simulink model "PMLSM_PI_FOC_Float_Baseline"  (R2026b)
settings: Solver=FixedStepDiscrete  StopTime=M1A_StopTime_s  FixedStep=Ts_Plant
InitFcn:
  | m1a_require_float_init(bdroot);
values from neighbouring files (symbols this model uses):
  Alignment_Enable = 0    [init_PMLSM_PI_FOC_Float_Baseline.m]
  Hold_Ticks = 30000    [init_PMLSM_PI_FOC_Float_Baseline.m]
  Host_AutoStart_EN = 1    [init_PMLSM_PI_FOC_Float_Baseline.m]
  Host_Close_Loop_EN = 1    [init_PMLSM_PI_FOC_Float_Baseline.m]
  Host_Id_A = 0    [init_PMLSM_PI_FOC_Float_Baseline.m]
  Host_Iq_A = 0    [init_PMLSM_PI_FOC_Float_Baseline.m]
  Host_Iq_Test_Mode = 0    [init_PMLSM_PI_FOC_Float_Baseline.m]
  Host_Load_N = 0    [init_PMLSM_PI_FOC_Float_Baseline.m]
  Host_Move_Request = 0    [init_PMLSM_PI_FOC_Float_Baseline.m]
  Host_PI_Reset_EN = 0    [init_PMLSM_PI_FOC_Float_Baseline.m]
  Host_Position_Loop_EN = 1    [init_PMLSM_PI_FOC_Float_Baseline.m]
  Host_PWM_EN = 1    [init_PMLSM_PI_FOC_Float_Baseline.m]
  Host_Ready_Ticks = 5    [init_PMLSM_PI_FOC_Float_Baseline.m]
  Host_Replay_EN = 0    [init_PMLSM_PI_FOC_Float_Baseline.m]
  Host_Speed_mmps = 0    [init_PMLSM_PI_FOC_Float_Baseline.m]
  Host_Speed_Ramp_s = 0.1    [init_PMLSM_PI_FOC_Float_Baseline.m]
  Host_Start_s = 0.05    [init_PMLSM_PI_FOC_Float_Baseline.m]
  Host_Target_mm = 10    [init_PMLSM_PI_FOC_Float_Baseline.m]
  Host_Traj_Amax = 100    [init_PMLSM_PI_FOC_Float_Baseline.m]
  Host_Traj_Jmax = 1000    [init_PMLSM_PI_FOC_Float_Baseline.m]
  Host_Traj_Vmax = 10    [init_PMLSM_PI_FOC_Float_Baseline.m]
  Id_Init_Step = Id_Init_Target/Ramp_Ticks    (= 5e-05)    [init_PMLSM_PI_FOC_Float_Baseline.m]
  Id_Init_Target = 0.5    [init_PMLSM_PI_FOC_Float_Baseline.m]
  Id_Release_Ramp_Ticks = 2000    [init_PMLSM_PI_FOC_Float_Baseline.m]
  Init_Reset = 0    [init_PMLSM_PI_FOC_Float_Baseline.m]
  Init_Start = 0    [init_PMLSM_PI_FOC_Float_Baseline.m]
  Iq_int_limit = 0.5    [init_PMLSM_PI_FOC_Float_Baseline.m]
  Kaw_d = Tuning_Gains.Kaw_d    [init_PMLSM_PI_FOC_Float_Baseline.m]
  Kaw_q = Tuning_Gains.Kaw_q    [init_PMLSM_PI_FOC_Float_Baseline.m]
  Kaw_s = Tuning_Gains.Kaw_s    [init_PMLSM_PI_FOC_Float_Baseline.m]
  Ki_ACR = Tuning_Gains.Ki_ACR    [init_PMLSM_PI_FOC_Float_Baseline.m]
  Ki_ASR = Tuning_Gains.Ki_ASR    [init_PMLSM_PI_FOC_Float_Baseline.m]
  Kp_ACR = Tuning_Gains.Kp_ACR    [init_PMLSM_PI_FOC_Float_Baseline.m]
  Kp_ASR = Tuning_Gains.Kp_ASR    [init_PMLSM_PI_FOC_Float_Baseline.m]
  Kp_pos = Tuning_Gains.Kp_pos    [init_PMLSM_PI_FOC_Float_Baseline.m]
  M1A_PWM_Update_Delay_s = T_pwm/2    (= 5e-05)    [init_PMLSM_PI_FOC_Float_Baseline.m]
  PMLSM_Bv_N_per_mps = 0    [init_PMLSM_PI_FOC_Float_Baseline.m]
  PMLSM_deadtime_current_eps_A = 1e-4    (= 0.0001)    [init_PMLSM_PI_FOC_Float_Baseline.m]
  PMLSM_deadtime_ratio = PMLSM_deadtime_s/T_pwm    (= 0.01)    [init_PMLSM_PI_FOC_Float_Baseline.m]
  PMLSM_Fc_N = 0    [init_PMLSM_PI_FOC_Float_Baseline.m]
  PMLSM_Kf_peak_N_per_Apeak = 31.4/sqrt(2)    [init_PMLSM_PI_FOC_Float_Baseline.m]
  PMLSM_Ld_H = 1.745e-3    (= 0.001745)    [init_PMLSM_PI_FOC_Float_Baseline.m]
  PMLSM_Lq_H = PMLSM_Ld_H    (= 0.001745)    [init_PMLSM_PI_FOC_Float_Baseline.m]
  PMLSM_M_kg = 0.91    [init_PMLSM_PI_FOC_Float_Baseline.m]
  PMLSM_psi_f_Wb = 0.141    [init_PMLSM_PI_FOC_Float_Baseline.m]
  PMLSM_Rs_ohm = 2.37    [init_PMLSM_PI_FOC_Float_Baseline.m]
  PMLSM_tau_NN_m = 0.06    [init_PMLSM_PI_FOC_Float_Baseline.m]
  PMLSM_theta_offset_rad = 0    [init_PMLSM_PI_FOC_Float_Baseline.m]
  PMLSM_Ts_s = Ts_Plant    (= 1e-06)    [init_PMLSM_PI_FOC_Float_Baseline.m]
  PMLSM_v_eps_mps = 1e-3    (= 0.001)    [init_PMLSM_PI_FOC_Float_Baseline.m]
  Pos_deadband = 0.02    [init_PMLSM_PI_FOC_Float_Baseline.m]
  Ramp_Ticks = 10000    [init_PMLSM_PI_FOC_Float_Baseline.m]
  Simulation_Travel_Fault = 0    [init_PMLSM_PI_FOC_Float_Baseline.m]
  Speed_loop_Iq_Limit = 1    [init_PMLSM_PI_FOC_Float_Baseline.m]
  T_pwm = 1e-4    (= 0.0001)    [init_PMLSM_PI_FOC_Float_Baseline.m]
  Tau_e_mm = PMLSM_tau_NN_m*1000    (= 60)    [init_PMLSM_PI_FOC_Float_Baseline.m]
  theta_align_const = 0    [init_PMLSM_PI_FOC_Float_Baseline.m]
  Theta_Offset_Fine = 0    [init_PMLSM_PI_FOC_Float_Baseline.m]
  Ts = Ts_ACR    (= 0.0001)    [init_PMLSM_PI_FOC_Float_Baseline.m]
  Ts_ACR = T_pwm    (= 0.0001)    [init_PMLSM_PI_FOC_Float_Baseline.m]
  Ts_ASR = 10*Ts_ACR    (= 0.001)    [init_PMLSM_PI_FOC_Float_Baseline.m]
  Ts_Plant = 1e-6    (= 1e-06)    [init_PMLSM_PI_FOC_Float_Baseline.m]
  Ts_POS = 10*Ts_ASR    (= 0.01)    [init_PMLSM_PI_FOC_Float_Baseline.m]
  Udc = 48    [init_PMLSM_PI_FOC_Float_Baseline.m]
  v_ff_eps = 0.5    [init_PMLSM_PI_FOC_Float_Baseline.m]
  v_over_eps = 3    [init_PMLSM_PI_FOC_Float_Baseline.m]
  V_pos_max_mmps = 20    [init_PMLSM_PI_FOC_Float_Baseline.m]
  v_ref_max = 20    [init_PMLSM_PI_FOC_Float_Baseline.m]
  v_ref_set_step_dn = v_ref_set_rate_dn*Ts_ACR    (= 0.005)    [init_PMLSM_PI_FOC_Float_Baseline.m]
  v_ref_set_step_up = v_ref_set_rate_up*Ts_ACR    (= 0.005)    [init_PMLSM_PI_FOC_Float_Baseline.m]
  v_ref_zero_eps = 0    [init_PMLSM_PI_FOC_Float_Baseline.m]
undefined symbols (not defined in the file or in its folder): DiscIntNeverNeededParam, Iq_fric_run, Iq_fric_start, v_stick_off, v_stick_on
libraries: simulink x7, mcbeeMathTransformLib x2
(part 1 of 2)
settings Model: Creator=lww  LastModifiedBy=lww
settings DataIOCC: SaveOutput=off  SaveTime=off

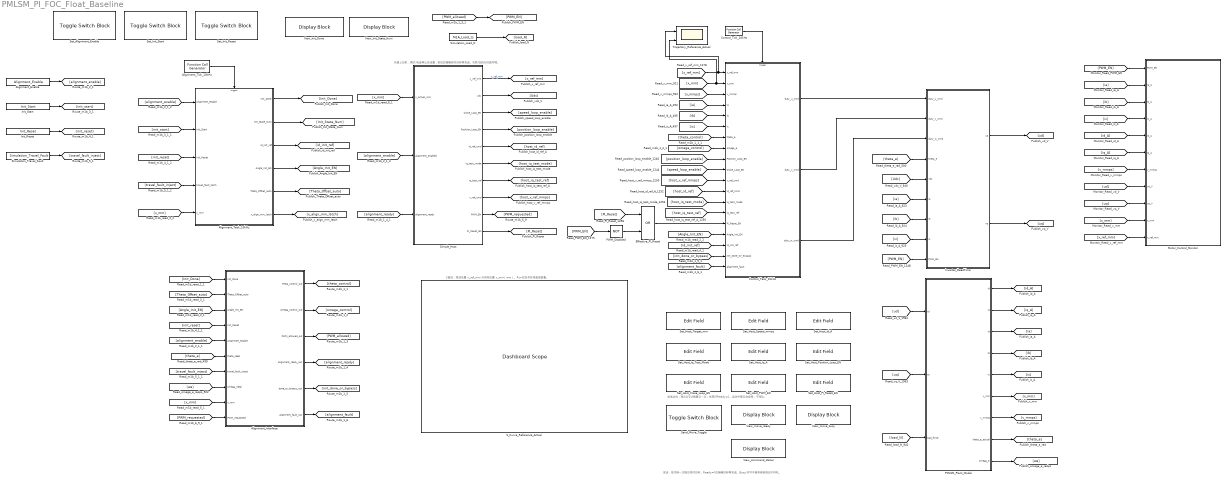
== system PMLSM_PI_FOC_Float_Baseline ==
  note: 仿真上位机：模式/轨迹停止后设置；到位后编辑绝对目标再发送。负载/母线为仿真环境。
  note: S曲线：规划位置 x_ref_mm 与实际位置 x_mm（mm）。Run后在本区域直接查看。
  note: 发送点位：每次0/1切换提交一次；先等待Ready=1，运动中提交会拒绝，不排队。
  note: 发送：每切换一次提交绝对目标；Ready=1后编辑目标再发送。Busy/对齐中请求被拒绝且不排队。
  Alignment_Enable : Constant  Value=Alignment_Enable  OutDataTypeStr=double  SampleTime=Ts_ACR
  Alignment_Interface : Subsystem
  Alignment_Task_10kHz : Subsystem
  Alignment_Tick_10kHz : FunctionCallGenerator  Priority=-100  SampleTime=Ts
  Control_Task_10kHz : Subsystem
  Control_Tick_10kHz : FunctionCallGenerator  Priority=100  SampleTime=Ts
  Effective_PI_Reset : Logic  Operator=OR  AllPortsSameDT=off  OutDataTypeStr=boolean
  Init_Reset : Constant  Value=Init_Reset  SampleTime=Ts_ACR
  Init_Start : Constant  Value=Init_Start  SampleTime=Ts_ACR
  Inverter_DeadTime : Subsystem
  Motor_Control_Monitor : Subsystem
  PMLSM_Plant_Model : Subsystem
  PWM_Disabled : Logic  Operator=NOT  AllPortsSameDT=off  OutDataTypeStr=boolean
  S_Curve_Reference_Actual : DashboardScope  FontColor=[0.0, 0.0, 0.0]
  Send_Move_Toggle : ToggleSwitchBlock
  Set_Alignment_Enable : ToggleSwitchBlock
  Set_Host_Close_Loop_EN : EditField  ShowInitialText=on  Alignment=Center
  Set_Host_Id_A : EditField  ShowInitialText=on  Alignment=Center
  Set_Host_Iq_A : EditField  ShowInitialText=on  Alignment=Center
  Set_Host_Iq_Test_Mode : EditField  ShowInitialText=on  Alignment=Center
  Set_Host_PI_Reset_EN : EditField  ShowInitialText=on  Alignment=Center
  Set_Host_PWM_EN : EditField  ShowInitialText=on  Alignment=Center
  Set_Host_Position_Loop_EN : EditField  ShowInitialText=on  Alignment=Center
  Set_Host_Speed_mmps : EditField  ShowInitialText=on  Alignment=Center
  Set_Host_Target_mm : EditField  ShowInitialText=on  Alignment=Center
  Set_Init_Reset : ToggleSwitchBlock
  Set_Init_Start : ToggleSwitchBlock
  Simple_Host : Subsystem
  Simulation_Load_N : FromWorkspace  VariableName=M1A_Load_ts  SampleTime=Ts_Plant  Interpolate=off  OutputAfterFinalValue=Holding final value
  Simulation_Travel_Fault : Constant  Value=Simulation_Travel_Fault  OutDataTypeStr=double  SampleTime=Ts_ACR
  Trajectory_Reference_Actual : Scope  NumInputPorts=2
      settings: ActiveDisplayYMinimum=0.99182264665726316  ActiveDisplayYMaximum=1.0007838303678565
  View_Init_Done : DisplayBlock  Transparency=1  GridColor=[0.502, 0.502, 0.502]
  View_Init_State_Num : DisplayBlock  Transparency=1  GridColor=[0.502, 0.502, 0.502]
  View_command_status : DisplayBlock  Transparency=1  GridColor=[0.502, 0.502, 0.502]
  View_move_busy : DisplayBlock  Transparency=1  GridColor=[0.502, 0.502, 0.502]
  View_move_ready : DisplayBlock  Transparency=1  GridColor=[0.502, 0.502, 0.502]
  wires:
  [PWM_EN] -> PWM_Disabled/1
  PWM_Disabled/1 -> Effective_PI_Reset/2
  Effective_PI_Reset/1 -> Control_Task_10kHz/15(PI_Reset_EN)
  [speed_loop_enable] -> Control_Task_10kHz/10(Close_Loop_EN)
  [position_loop_enable] -> Control_Task_10kHz/9(Position_Loop_EN)
  [host_v_ref_mmps] -> Control_Task_10kHz/11(v_ref_cmd)
  [host_id_ref] -> Control_Task_10kHz/12(id_ref_cmd)
  [host_iq_test_mode] -> Control_Task_10kHz/13(iq_test_mode)
  [host_iq_test_ref] -> Control_Task_10kHz/14(iq_test_ref)
  [PI_Reset] -> Effective_PI_Reset/1
  [x_mm] -> Trajectory_Reference_Actual/2, Control_Task_10kHz/2(x_mm)
  [v_mmps] -> Control_Task_10kHz/3(v_mmps)
  [ia] -> Control_Task_10kHz/4(ia)
  [ib] -> Control_Task_10kHz/5(ib)
  [ic] -> Control_Task_10kHz/6(ic)
  [x_ref_mm] -> Trajectory_Reference_Actual/1, Control_Task_10kHz/1(x_ref_mm)
  PMLSM_Plant_Model/6(x_mm) -> [x_mm]
  PMLSM_Plant_Model/7(v_mmps) -> [v_mmps]
  PMLSM_Plant_Model/3(ia) -> [ia]
  PMLSM_Plant_Model/4(ib) -> [ib]
  PMLSM_Plant_Model/5(ic) -> [ic]
  PMLSM_Plant_Model/8(theta_e_actual) -> [theta_e]
  PMLSM_Plant_Model/9(omega_e) -> [we]
  PMLSM_Plant_Model/1(id) -> [id_A]
  PMLSM_Plant_Model/2(iq) -> [iq_A]
  [load_N] -> PMLSM_Plant_Model/3(load_force)
  [uq] -> PMLSM_Plant_Model/2(vq)
  [ud] -> PMLSM_Plant_Model/1(vd)
  [ic] -> Inverter_DeadTime/8(ic)
  [ib] -> Inverter_DeadTime/7(ib)
  [ia] -> Inverter_DeadTime/6(ia)
  [theta_e] -> Inverter_DeadTime/4(theta_e)
  [Udc] -> Inverter_DeadTime/5(vdc)
  Inverter_DeadTime/1(vd) -> [ud]
  Inverter_DeadTime/2(vq) -> [uq]
  [PWM_EN] -> Inverter_DeadTime/9(PWM_EN)
  Control_Task_10kHz/1(duty_u_cmd) -> Inverter_DeadTime/1(duty_u_cmd)
  Control_Task_10kHz/2(duty_v_cmd) -> Inverter_DeadTime/2(duty_v_cmd)
  Control_Task_10kHz/3(duty_w_cmd) -> Inverter_DeadTime/3(duty_w_cmd)
  Simulation_Load_N/1 -> [load_N]
  Simple_Host/1(x_ref_mm) -> [x_ref_mm]  "x_ref_mm"
  Simple_Host/2(vdc) -> [Udc]
  Simple_Host/3(Close_Loop_EN) -> [speed_loop_enable]
  Simple_Host/4(Position_Loop_EN) -> [position_loop_enable]
  Simple_Host/5(id_ref_cmd) -> [host_id_ref]
  Simple_Host/6(iq_test_mode) -> [host_iq_test_mode]
  Simple_Host/7(iq_test_ref) -> [host_iq_test_ref]
  Simple_Host/8(v_ref_cmd) -> [host_v_ref_mmps]
  Simple_Host/10(PI_Reset_EN) -> [PI_Reset]
  [PWM_EN] -> Motor_Control_Monitor/1(PWM_EN)
  [ia] -> Motor_Control_Monitor/2(ia_A)
  [ib] -> Motor_Control_Monitor/3(ib_A)
  [ic] -> Motor_Control_Monitor/4(ic_A)
  [id_A] -> Motor_Control_Monitor/5(id_A)
  [iq_A] -> Motor_Control_Monitor/6(iq_A)
  [v_mmps] -> Motor_Control_Monitor/7(v_mmps)
  [ud] -> Motor_Control_Monitor/8(vd_V)
  [uq] -> Motor_Control_Monitor/9(vq_V)
  [x_mm] -> Motor_Control_Monitor/10(x_mm)
  [x_ref_mm] -> Motor_Control_Monitor/11(x_ref_mm)
  Alignment_Task_10kHz/1(Init_Done) -> [Init_Done]
  Alignment_Task_10kHz/2(Init_State_Num) -> [Init_State_Num]
  Alignment_Task_10kHz/3(id_init_ref) -> [id_init_ref]
  Alignment_Task_10kHz/4(Angle_Init_EN) -> [Angle_Init_EN]
  Alignment_Task_10kHz/5(Theta_Offset_auto) -> [Theta_Offset_auto]
  Alignment_Task_10kHz/6(x_align_mm_latch) -> [x_align_mm_latch]
  Alignment_Tick_10kHz/1 -> Alignment_Task_10kHz/Trigger
  Control_Tick_10kHz/1 -> Control_Task_10kHz/Trigger
  [theta_e] -> Alignment_Interface/6(theta_ideal)
  [we] -> Alignment_Interface/8(omega_ideal)
  Alignment_Interface/1(theta_control_out) -> [theta_control]
  [theta_control] -> Control_Task_10kHz/7(theta_e)
  Alignment_Interface/2(omega_control_out) -> [omega_control]
  [omega_control] -> Control_Task_10kHz/8(omega_e)
  Alignment_Interface/3(PWM_allowed_out) -> [PWM_allowed]
  [PWM_allowed] -> [PWM_EN]
  Alignment_Interface/4(alignment_ready_out) -> [alignment_ready]
  [alignment_ready] -> Simple_Host/3(alignment_ready)
  Alignment_Interface/5(done_or_bypass_out) -> [init_done_or_bypass]
  [init_done_or_bypass] -> Control_Task_10kHz/18(Init_Done_Or_Bypass)
  Alignment_Interface/6(alignment_fault_out) -> [alignment_fault]
  [alignment_fault] -> Control_Task_10kHz/19(alignment_fault)
  Alignment_Enable/1 -> [alignment_enable]
  [alignment_enable] -> Alignment_Interface/5(Alignment_Enable)
  [alignment_enable] -> Alignment_Task_10kHz/1(Alignment_Enable)
  [alignment_enable] -> Simple_Host/2(alignment_enabled)
  Init_Start/1 -> [init_start]
  [init_start] -> Alignment_Task_10kHz/2(Init_Start)
  Init_Reset/1 -> [init_reset]
  [init_reset] -> Alignment_Interface/4(Init_Reset)
  [init_reset] -> Alignment_Task_10kHz/3(Init_Reset)
  Simulation_Travel_Fault/1 -> [travel_fault_inject]
  [travel_fault_inject] -> Alignment_Interface/7(travel_fault_inject)
  [travel_fault_inject] -> Alignment_Task_10kHz/4(travel_fault_latch)
  Simple_Host/9(PWM_EN) -> [PWM_requested]
  [PWM_requested] -> Alignment_Interface/10(PWM_requested)
  [Init_Done] -> Alignment_Interface/1(Init_Done)
  [Angle_Init_EN] -> Alignment_Interface/3(Angle_Init_EN)
  [Angle_Init_EN] -> Control_Task_10kHz/16(Angle_Init_EN)
  [Theta_Offset_auto] -> Alignment_Interface/2(Theta_Offset_auto)
  [id_init_ref] -> Control_Task_10kHz/17(id_init_ref)
  [x_mm] -> Alignment_Interface/9(x_mm)
  [x_mm] -> Alignment_Task_10kHz/5(x_mm)
  [x_mm] -> Simple_Host/1(x_actual_mm)

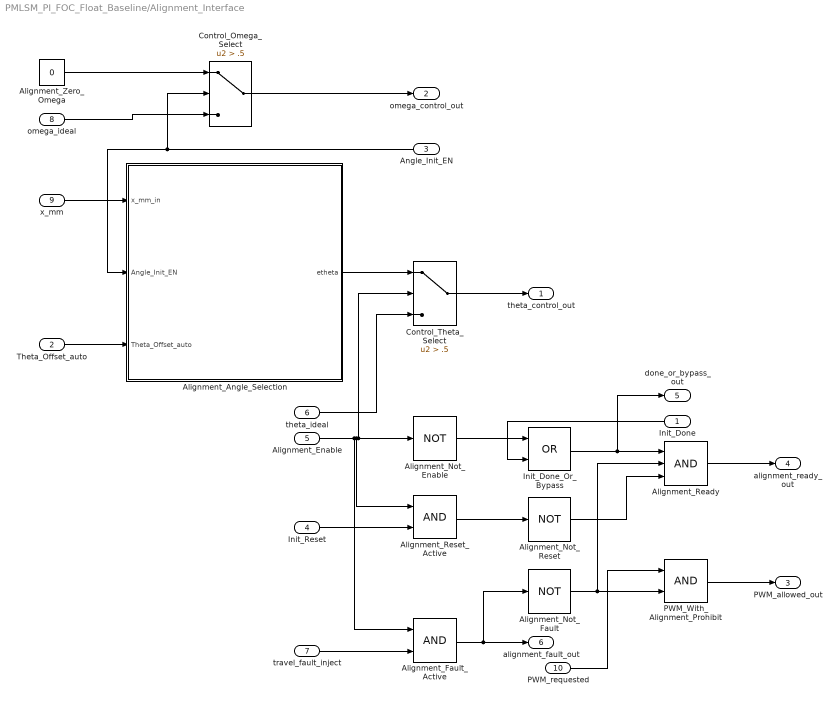
== system PMLSM_PI_FOC_Float_Baseline/Alignment_Interface ==
  Init_Done : Inport
  Theta_Offset_auto : Inport  Port=2
  Angle_Init_EN : Inport  Port=3
  Init_Reset : Inport  Port=4
  Alignment_Enable : Inport  Port=5
  theta_ideal : Inport  Port=6
  travel_fault_inject : Inport  Port=7
  omega_ideal : Inport  Port=8
  x_mm : Inport  Port=9
  PWM_requested : Inport  Port=10
  Alignment_Angle_Selection : Subsystem
  Alignment_Fault_Active : Logic  AllPortsSameDT=off  OutDataTypeStr=boolean
  Alignment_Not_Enable : Logic  Operator=NOT  AllPortsSameDT=off  OutDataTypeStr=boolean
  Alignment_Not_Fault : Logic  Operator=NOT  AllPortsSameDT=off  OutDataTypeStr=boolean
  Alignment_Not_Reset : Logic  Operator=NOT  AllPortsSameDT=off  OutDataTypeStr=boolean
  Alignment_Ready : Logic  Inputs=3  AllPortsSameDT=off  OutDataTypeStr=boolean
  Alignment_Reset_Active : Logic  AllPortsSameDT=off  OutDataTypeStr=boolean
  Alignment_Zero_Omega : Constant  Value=0
  Control_Omega_Select : Switch  Criteria=u2 > Threshold  Threshold=.5
  Control_Theta_Select : Switch  Criteria=u2 > Threshold  Threshold=.5
  Init_Done_Or_Bypass : Logic  Operator=OR  AllPortsSameDT=off  OutDataTypeStr=boolean
  PWM_With_Alignment_Prohibit : Logic  AllPortsSameDT=off  OutDataTypeStr=boolean
  theta_control_out : Outport
  omega_control_out : Outport  Port=2
  PWM_allowed_out : Outport  Port=3
  alignment_ready_out : Outport  Port=4
  done_or_bypass_out : Outport  Port=5
  alignment_fault_out : Outport  Port=6
  wires:
  Init_Done/1 -> Init_Done_Or_Bypass/2
  Alignment_Zero_Omega/1 -> Control_Omega_Select/1
  omega_ideal/1 -> Control_Omega_Select/3
  Alignment_Not_Enable/1 -> Init_Done_Or_Bypass/1
  Alignment_Enable/1 -> Alignment_Not_Enable/1, Control_Theta_Select/2, Alignment_Reset_Active/1, Alignment_Fault_Active/1
  x_mm/1 -> Alignment_Angle_Selection/1(x_mm_in)
  Alignment_Ready/1 -> alignment_ready_out/1
  Alignment_Angle_Selection/1(etheta) -> Control_Theta_Select/1
  Theta_Offset_auto/1 -> Alignment_Angle_Selection/3(Theta_Offset_auto)
  Control_Omega_Select/1 -> omega_control_out/1
  theta_ideal/1 -> Control_Theta_Select/3
  Init_Reset/1 -> Alignment_Reset_Active/2
  travel_fault_inject/1 -> Alignment_Fault_Active/2
  Angle_Init_EN/1 -> Control_Omega_Select/2, Alignment_Angle_Selection/2(Angle_Init_EN)
  Control_Theta_Select/1 -> theta_control_out/1
  Alignment_Reset_Active/1 -> Alignment_Not_Reset/1
  Alignment_Fault_Active/1 -> Alignment_Not_Fault/1, alignment_fault_out/1
  Init_Done_Or_Bypass/1 -> done_or_bypass_out/1, Alignment_Ready/1
  Alignment_Not_Reset/1 -> Alignment_Ready/3
  Alignment_Not_Fault/1 -> Alignment_Ready/2, PWM_With_Alignment_Prohibit/2
  PWM_requested/1 -> PWM_With_Alignment_Prohibit/1
  PWM_With_Alignment_Prohibit/1 -> PWM_allowed_out/1

== system PMLSM_PI_FOC_Float_Baseline/Alignment_Task_10kHz ==
  Alignment_Enable : Inport
  Init_Start : Inport  Port=2
  Init_Reset : Inport  Port=3
  travel_fault_latch : Inport  Port=4
  x_mm : Inport  Port=5
  Tick : TriggerPort  TriggerType=function-call  VariantControl=(inherit)
  Enabled_Original_MIL : Subsystem
  Init_Done : Outport
  Init_State_Num : Outport  Port=2
  id_init_ref : Outport  Port=3
  Angle_Init_EN : Outport  Port=4
  Theta_Offset_auto : Outport  Port=5
  x_align_mm_latch : Outport  Port=6
  wires:
  Alignment_Enable/1 -> Enabled_Original_MIL/Enable
  Enabled_Original_MIL/2(Init_State_Num) -> Init_State_Num/1
  Init_Start/1 -> Enabled_Original_MIL/1(Init_Start)
  Enabled_Original_MIL/3(id_init_ref) -> id_init_ref/1
  Init_Reset/1 -> Enabled_Original_MIL/2(Init_Reset)
  travel_fault_latch/1 -> Enabled_Original_MIL/3(travel_fault_latch)
  x_mm/1 -> Enabled_Original_MIL/4(x_mm)
  Enabled_Original_MIL/1(Init_Done) -> Init_Done/1
  Enabled_Original_MIL/4(Angle_Init_EN) -> Angle_Init_EN/1
  Enabled_Original_MIL/5(Theta_Offset_auto) -> Theta_Offset_auto/1
  Enabled_Original_MIL/6(x_align_mm_latch) -> x_align_mm_latch/1

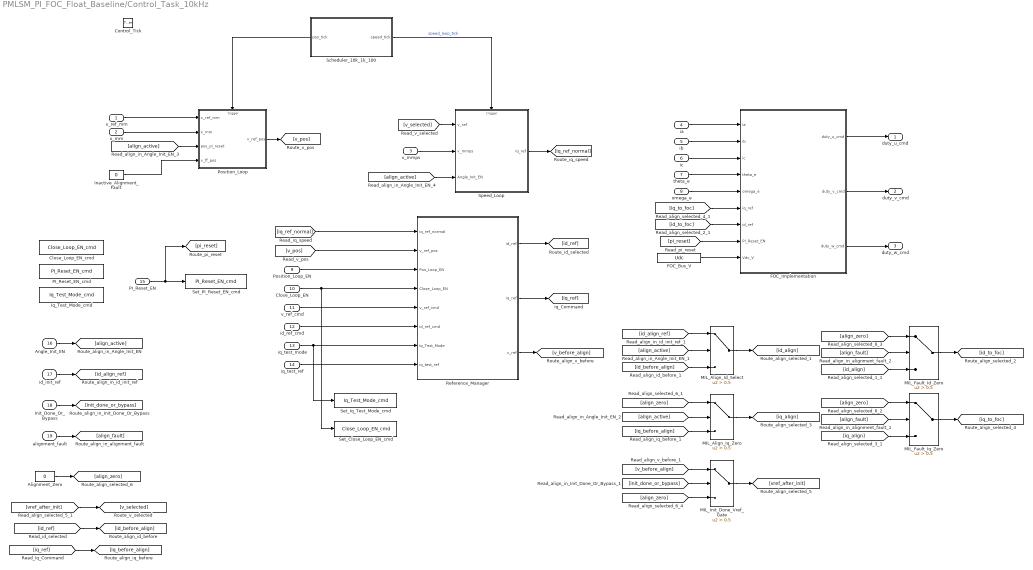
== system PMLSM_PI_FOC_Float_Baseline/Control_Task_10kHz ==
  x_ref_mm : Inport
  x_mm : Inport  Port=2
  v_mmps : Inport  Port=3
  ia : Inport  Port=4
  ib : Inport  Port=5
  ic : Inport  Port=6
  theta_e : Inport  Port=7
  omega_e : Inport  Port=8
  Position_Loop_EN : Inport  Port=9
  Close_Loop_EN : Inport  Port=10
  v_ref_cmd : Inport  Port=11
  id_ref_cmd : Inport  Port=12
  iq_test_mode : Inport  Port=13
  iq_test_ref : Inport  Port=14
  PI_Reset_EN : Inport  Port=15
  Angle_Init_EN : Inport  Port=16
  id_init_ref : Inport  Port=17
  Init_Done_Or_Bypass : Inport  Port=18
  alignment_fault : Inport  Port=19
  Control_Tick : TriggerPort  TriggerType=function-call  VariantControl=(inherit)  PortDimensions=1
  Alignment_Zero : Constant  Value=0
  Close_Loop_EN_cmd : DataStoreMemory  DataStoreName=Close_Loop_EN_cmd  WriteAfterWriteMsg=warning  InitialValue=1  ShowAdditionalParam=off
  FOC_Bus_V : Constant  Value=Udc  SampleTime=-1
  FOC_Implementation : Subsystem  Variant=on  EmptyChoice=on
  Inactive_Alignment_Fault : Constant  Value=0
  Iq_Test_Mode_cmd : DataStoreMemory  DataStoreName=Iq_Test_Mode_cmd  WriteAfterWriteMsg=warning  ShowAdditionalParam=off
  MIL_Align_Id_Select : Switch  Criteria=u2 > Threshold  Threshold=0.5  SaturateOnIntegerOverflow=off  InputSameDT=off
  MIL_Align_Iq_Zero : Switch  Criteria=u2 > Threshold  Threshold=0.5  SaturateOnIntegerOverflow=off  InputSameDT=off
  MIL_Fault_Id_Zero : Switch  Criteria=u2 > Threshold  Threshold=0.5  SaturateOnIntegerOverflow=off  InputSameDT=off
  MIL_Fault_Iq_Zero : Switch  Criteria=u2 > Threshold  Threshold=0.5  SaturateOnIntegerOverflow=off  InputSameDT=off
  MIL_Init_Done_Vref_Gate : Switch  Criteria=u2 > Threshold  Threshold=0.5  SaturateOnIntegerOverflow=off  InputSameDT=off
  PI_Reset_EN_cmd : DataStoreMemory  DataStoreName=PI_Reset_EN_cmd  WriteAfterWriteMsg=warning  ShowAdditionalParam=off
  Position_Loop : Subsystem  TreatAsAtomicUnit=on
  Reference_Manager : Subsystem
  Scheduler_10k_1k_100 : Subsystem
      settings: PortSchema="{\"entries\":[{\"content\":{\"sides\":[{\"content\":{\"connectorIds\":[\"Out2\"]},\"type\":\"ConnectorPlacement.EquallySpacedRectSide\",\"uuid\":\"7a2cd2ad-1b6d-4ced-b4c0-dea2e76e4441\"},{\"content\":{\"connectorIds\":[\"Out1\"],\"side\":\"RIGHT\"},\"type\":\"ConnectorPlacement.EquallySpacedRectSide\",\"uuid\":\"f7db3b94-1126-4089-83bd-8e57d20e6fd7\"},{\"content\":{\"side\":\"TOP\"},\"type\":\"ConnectorPlacement.EquallySpacedRectSide\",\"uuid\":\"9153f6b5-22af-48be-92c0-68be43f93648\"}]},\"type\":\"ConnectorPlacement.EquallySpacedConnector\",\"uuid\":\"029fb485-bddc-4cd2-9c64-7547c8dffd2b\"}],\"packageUris\":[\"http://schema.mathworks.com/mf0/Connector/R2020b\"],\"version\":\"1.0\"}"
  Set_Close_Loop_EN_cmd : DataStoreWrite  Priority=-10  DataStoreName=Close_Loop_EN_cmd  IndexOptions=Index vector (dialog)  Indices=1  OutputSizes=1
  Set_Iq_Test_Mode_cmd : DataStoreWrite  Priority=-10  DataStoreName=Iq_Test_Mode_cmd  IndexOptions=Index vector (dialog)  Indices=1  OutputSizes=1
  Set_PI_Reset_EN_cmd : DataStoreWrite  Priority=-10  DataStoreName=PI_Reset_EN_cmd  IndexOptions=Index vector (dialog)  Indices=1  OutputSizes=1
  Speed_Loop : Subsystem  TreatAsAtomicUnit=on
  duty_u_cmd : Outport
  duty_v_cmd : Outport  Port=2
  duty_w_cmd : Outport  Port=3
  wires:
  iq_test_ref/1 -> Reference_Manager/8(iq_test_ref)
  id_ref_cmd/1 -> Reference_Manager/6(id_ref_cmd)
  v_ref_cmd/1 -> Reference_Manager/5(v_ref_cmd)
  Position_Loop_EN/1 -> Reference_Manager/3(Pos_Loop_EN)
  [v_selected] -> Speed_Loop/1(v_ref)
  [iq_ref_normal] -> Reference_Manager/1(iq_ref_normal)
  [v_pos] -> Reference_Manager/2(v_ref_pos)
  Inactive_Alignment_Fault/1 -> Position_Loop/4(v_ff_pos)
  Speed_Loop/1(iq_ref) -> [iq_ref_normal]
  Position_Loop/1(v_ref_pos) -> [v_pos]
  x_mm/1 -> Position_Loop/2(x_mm)
  x_ref_mm/1 -> Position_Loop/1(x_ref_mm)
  Scheduler_10k_1k_100/1(speed_tick) -> Speed_Loop/Trigger  "speed_loop_tick"
  Scheduler_10k_1k_100/2(pos_tick) -> Position_Loop/Trigger
  PI_Reset_EN/1 -> [pi_reset], Set_PI_Reset_EN_cmd/1
  iq_test_mode/1 -> Set_Iq_Test_Mode_cmd/1, Reference_Manager/7(Iq_Test_Mode)
  Close_Loop_EN/1 -> Set_Close_Loop_EN_cmd/1, Reference_Manager/4(Close_Loop_EN)
  v_mmps/1 -> Speed_Loop/2(v_mmps)
  Reference_Manager/1(id_ref) -> [id_ref]
  Reference_Manager/2(iq_ref) -> [iq_ref]
  MIL_Align_Id_Select/1 -> [id_align]
  [id_align] -> MIL_Fault_Id_Zero/3
  MIL_Fault_Id_Zero/1 -> [id_to_foc]
  MIL_Align_Iq_Zero/1 -> [iq_align]
  [iq_align] -> MIL_Fault_Iq_Zero/3
  MIL_Fault_Iq_Zero/1 -> [iq_to_foc]
  MIL_Init_Done_Vref_Gate/1 -> [vref_after_init]
  [vref_after_init] -> [v_selected]
  Alignment_Zero/1 -> [align_zero]
  [align_zero] -> MIL_Align_Iq_Zero/1
  [align_zero] -> MIL_Fault_Iq_Zero/1
  [align_zero] -> MIL_Fault_Id_Zero/1
  [align_zero] -> MIL_Init_Done_Vref_Gate/3
  Angle_Init_EN/1 -> [align_active]
  [align_active] -> MIL_Align_Id_Select/2
  [align_active] -> MIL_Align_Iq_Zero/2
  [align_active] -> Position_Loop/3(pos_pi_reset)
  [align_active] -> Speed_Loop/3(Angle_Init_EN)
  id_init_ref/1 -> [id_align_ref]
  [id_align_ref] -> MIL_Align_Id_Select/1
  Init_Done_Or_Bypass/1 -> [init_done_or_bypass]
  [init_done_or_bypass] -> MIL_Init_Done_Vref_Gate/2
  alignment_fault/1 -> [align_fault]
  [align_fault] -> MIL_Fault_Iq_Zero/2
  [align_fault] -> MIL_Fault_Id_Zero/2
  [id_ref] -> [id_before_align]
  [id_before_align] -> MIL_Align_Id_Select/3
  [iq_ref] -> [iq_before_align]
  [iq_before_align] -> MIL_Align_Iq_Zero/3
  Reference_Manager/3(v_ref) -> [v_before_align]
  [v_before_align] -> MIL_Init_Done_Vref_Gate/1
  ia/1 -> FOC_Implementation/1(ia)
  ib/1 -> FOC_Implementation/2(ib)
  ic/1 -> FOC_Implementation/3(ic)
  theta_e/1 -> FOC_Implementation/4(theta_e)
  omega_e/1 -> FOC_Implementation/5(omega_e)
  [iq_to_foc] -> FOC_Implementation/6(iq_ref)
  [id_to_foc] -> FOC_Implementation/7(id_ref)
  [pi_reset] -> FOC_Implementation/8(PI_Reset_EN)
  FOC_Implementation/1(duty_u_cmd) -> duty_u_cmd/1
  FOC_Implementation/2(duty_v_cmd) -> duty_v_cmd/1
  FOC_Implementation/3(duty_w_cmd) -> duty_w_cmd/1
  FOC_Bus_V/1 -> FOC_Implementation/9(Vdc_V)

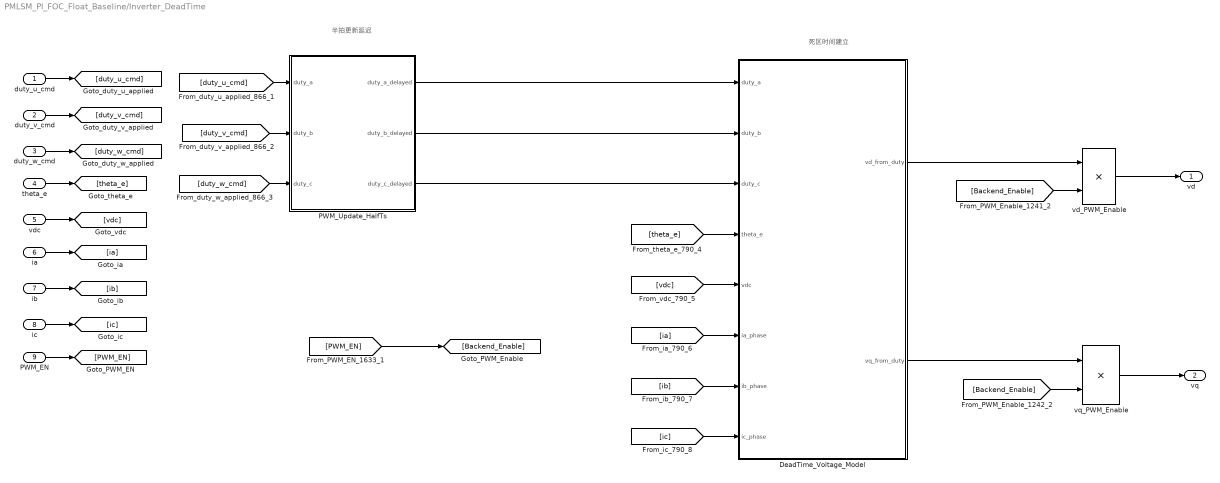
== system PMLSM_PI_FOC_Float_Baseline/Inverter_DeadTime ==
  note: 死区时间建立
  note: 半拍更新延迟
  duty_u_cmd : Inport
  duty_v_cmd : Inport  Port=2
  duty_w_cmd : Inport  Port=3
  theta_e : Inport  Port=4
  vdc : Inport  Port=5
  ia : Inport  Port=6
  ib : Inport  Port=7
  ic : Inport  Port=8
  PWM_EN : Inport  Port=9
  DeadTime_Voltage_Model : Subsystem
  PWM_Update_HalfTs : Subsystem
  vd_PWM_Enable : Product  Inputs=**
  vq_PWM_Enable : Product  Inputs=**
  vd : Outport
  vq : Outport  Port=2
  wires:
  [PWM_EN] -> [Backend_Enable]
  [ic] -> DeadTime_Voltage_Model/8(ic_phase)
  [ib] -> DeadTime_Voltage_Model/7(ib_phase)
  [ia] -> DeadTime_Voltage_Model/6(ia_phase)
  [vdc] -> DeadTime_Voltage_Model/5(vdc)
  [theta_e] -> DeadTime_Voltage_Model/4(theta_e)
  [duty_w_cmd] -> PWM_Update_HalfTs/3(duty_c)
  [duty_v_cmd] -> PWM_Update_HalfTs/2(duty_b)
  [duty_u_cmd] -> PWM_Update_HalfTs/1(duty_a)
  PWM_EN/1 -> [PWM_EN]
  PWM_Update_HalfTs/3(duty_c_delayed) -> DeadTime_Voltage_Model/3(duty_c)
  PWM_Update_HalfTs/2(duty_b_delayed) -> DeadTime_Voltage_Model/2(duty_b)
  PWM_Update_HalfTs/1(duty_a_delayed) -> DeadTime_Voltage_Model/1(duty_a)
  ic/1 -> [ic]
  ib/1 -> [ib]
  ia/1 -> [ia]
  vdc/1 -> [vdc]
  theta_e/1 -> [theta_e]
  duty_u_cmd/1 -> [duty_u_cmd]
  duty_v_cmd/1 -> [duty_v_cmd]
  duty_w_cmd/1 -> [duty_w_cmd]
  [Backend_Enable] -> vd_PWM_Enable/2
  [Backend_Enable] -> vq_PWM_Enable/2
  DeadTime_Voltage_Model/1(vd_from_duty) -> vd_PWM_Enable/1
  DeadTime_Voltage_Model/2(vq_from_duty) -> vq_PWM_Enable/1
  vd_PWM_Enable/1 -> vd/1
  vq_PWM_Enable/1 -> vq/1

== system PMLSM_PI_FOC_Float_Baseline/Motor_Control_Monitor ==
  PWM_EN : Inport
  ia_A : Inport  Port=2
  ib_A : Inport  Port=3
  ic_A : Inport  Port=4
  id_A : Inport  Port=5
  iq_A : Inport  Port=6
  v_mmps : Inport  Port=7
  vd_V : Inport  Port=8
  vq_V : Inport  Port=9
  x_mm : Inport  Port=10
  x_ref_mm : Inport  Port=11
  View_PWM_EN : Scope
  View_ia_A : Scope
  View_ib_A : Scope
  View_ic_A : Scope
  View_id_A : Scope
  View_iq_A : Scope
  View_v_mmps : Scope
  View_vd_V : Scope
  View_vq_V : Scope
  View_x_mm : Scope
  View_x_ref_mm : Scope
  wires:
  PWM_EN/1 -> View_PWM_EN/1
  ia_A/1 -> View_ia_A/1
  ib_A/1 -> View_ib_A/1
  ic_A/1 -> View_ic_A/1
  id_A/1 -> View_id_A/1
  iq_A/1 -> View_iq_A/1
  v_mmps/1 -> View_v_mmps/1
  vd_V/1 -> View_vd_V/1
  vq_V/1 -> View_vq_V/1
  x_mm/1 -> View_x_mm/1
  x_ref_mm/1 -> View_x_ref_mm/1

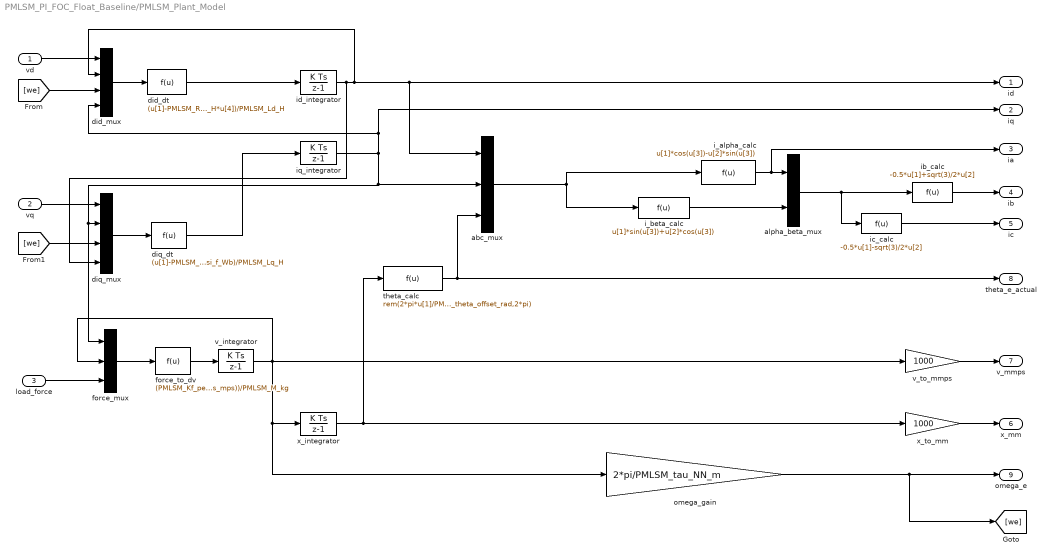
== system PMLSM_PI_FOC_Float_Baseline/PMLSM_Plant_Model ==
  vd : Inport
  vq : Inport  Port=2
  load_force : Inport  Port=3
  abc_mux : Mux  Inputs=3
  alpha_beta_mux : Mux  Inputs=2
  did_dt : Fcn  Expr=(u[1]-PMLSM_Rs_ohm*u[2]+u[3]*PMLSM_Lq_H*u[4])/PMLSM_Ld_H
  did_mux : Mux
  diq_dt : Fcn  Expr=(u[1]-PMLSM_Rs_ohm*u[2]-u[3]*PMLSM_Ld_H*u[4]-u[3]*PMLSM_psi_f_Wb)/PMLSM_Lq_H
  diq_mux : Mux
  force_mux : Mux  Inputs=3
  force_to_dv : Fcn  Expr=(PMLSM_Kf_peak_N_per_Apeak*u[1]-u[3]-PMLSM_Bv_N_per_mps*u[2]-PMLSM_Fc_N*tanh(u[2]/PMLSM_v_eps_mps))/PMLSM_M_kg
  i_alpha_calc : Fcn  Expr=u[1]*cos(u[3])-u[2]*sin(u[3])
  i_beta_calc : Fcn  Expr=u[1]*sin(u[3])+u[2]*cos(u[3])
  ib_calc : Fcn  Expr=-0.5*u[1]+sqrt(3)/2*u[2]
  ic_calc : Fcn  Expr=-0.5*u[1]-sqrt(3)/2*u[2]
  id_integrator : DiscreteIntegrator  gainval=1  SampleTime=PMLSM_Ts_s  ICPrevOutput=DiscIntNeverNeededParam  ICPrevScaledInput=DiscIntNeverNeededParam
  iq_integrator : DiscreteIntegrator  gainval=1  SampleTime=PMLSM_Ts_s  ICPrevOutput=DiscIntNeverNeededParam  ICPrevScaledInput=DiscIntNeverNeededParam
  omega_gain : Gain  Gain=2*pi/PMLSM_tau_NN_m
  theta_calc : Fcn  Expr=rem(2*pi*u[1]/PMLSM_tau_NN_m+PMLSM_theta_offset_rad,2*pi)
  v_integrator : DiscreteIntegrator  gainval=1  SampleTime=PMLSM_Ts_s  ICPrevOutput=DiscIntNeverNeededParam  ICPrevScaledInput=DiscIntNeverNeededParam
  v_to_mmps : Gain  Gain=1000
  x_integrator : DiscreteIntegrator  gainval=1  SampleTime=PMLSM_Ts_s  ICPrevOutput=DiscIntNeverNeededParam  ICPrevScaledInput=DiscIntNeverNeededParam
  x_to_mm : Gain  Gain=1000
  id : Outport
  iq : Outport  Port=2
  ia : Outport  Port=3
  ib : Outport  Port=4
  ic : Outport  Port=5
  x_mm : Outport  Port=6
  v_mmps : Outport  Port=7
  theta_e_actual : Outport  Port=8
  omega_e : Outport  Port=9
  wires:
  ic_calc/1 -> ic/1
  ib_calc/1 -> ib/1
  alpha_beta_mux/1 -> ic_calc/1, ib_calc/1
  i_beta_calc/1 -> alpha_beta_mux/2
  i_alpha_calc/1 -> alpha_beta_mux/1, ia/1
  force_to_dv/1 -> v_integrator/1
  force_mux/1 -> force_to_dv/1
  load_force/1 -> force_mux/3
  diq_dt/1 -> iq_integrator/1
  diq_mux/1 -> diq_dt/1
  vq/1 -> diq_mux/1
  did_dt/1 -> id_integrator/1
  did_mux/1 -> did_dt/1
  vd/1 -> did_mux/1
  x_to_mm/1 -> x_mm/1
  v_to_mmps/1 -> v_mmps/1
  theta_calc/1 -> theta_e_actual/1, abc_mux/3
  omega_gain/1 -> [we], omega_e/1
  id_integrator/1 -> id/1, abc_mux/1, did_mux/2, diq_mux/4
  iq_integrator/1 -> abc_mux/2, force_mux/1, diq_mux/2, iq/1, did_mux/4
  v_integrator/1 -> omega_gain/1, x_integrator/1, v_to_mmps/1, force_mux/2
  x_integrator/1 -> theta_calc/1, x_to_mm/1
  abc_mux/1 -> i_alpha_calc/1, i_beta_calc/1
  [we] -> did_mux/3
  [we] -> diq_mux/3

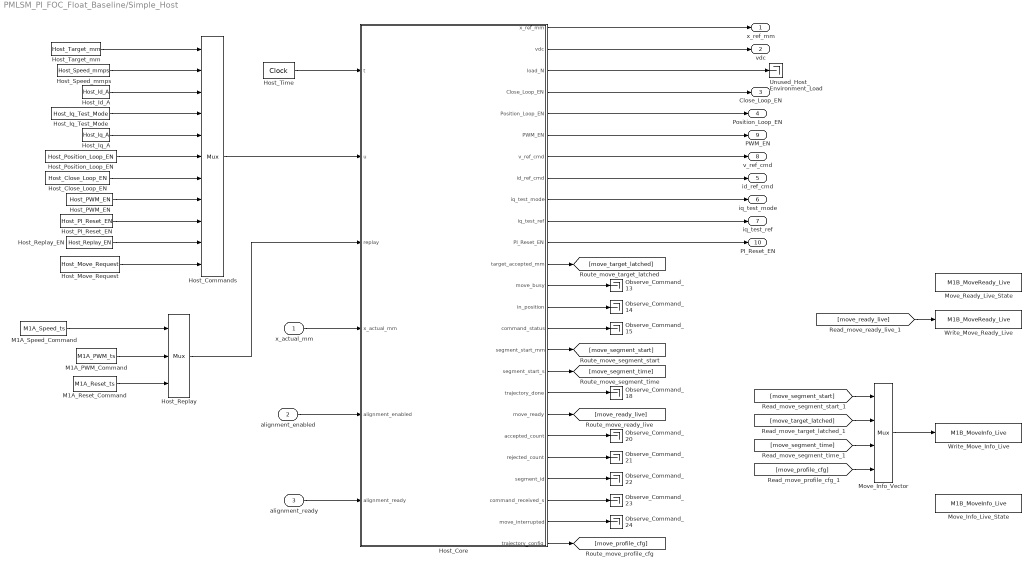
== system PMLSM_PI_FOC_Float_Baseline/Simple_Host ==
  x_actual_mm : Inport
  alignment_enabled : Inport  Port=2
  alignment_ready : Inport  Port=3
  Host_Close_Loop_EN : Constant  Value=Host_Close_Loop_EN  SampleTime=Ts_ACR
  Host_Commands : Mux  Inputs=11
  Host_Core : MATLAB Function  TreatAsAtomicUnit=on
  Host_Id_A : Constant  Value=Host_Id_A  SampleTime=Ts_ACR
  Host_Iq_A : Constant  Value=Host_Iq_A  SampleTime=Ts_ACR
  Host_Iq_Test_Mode : Constant  Value=Host_Iq_Test_Mode  SampleTime=Ts_ACR
  Host_Move_Request : Constant  Value=Host_Move_Request  SampleTime=Ts_ACR
  Host_PI_Reset_EN : Constant  Value=Host_PI_Reset_EN  SampleTime=Ts_ACR
  Host_PWM_EN : Constant  Value=Host_PWM_EN  SampleTime=Ts_ACR
  Host_Position_Loop_EN : Constant  Value=Host_Position_Loop_EN  SampleTime=Ts_ACR
  Host_Replay : Mux  Inputs=3
  Host_Replay_EN : Constant  Value=Host_Replay_EN  SampleTime=Ts_ACR
  Host_Speed_mmps : Constant  Value=Host_Speed_mmps  SampleTime=Ts_ACR
  Host_Target_mm : Constant  Value=Host_Target_mm  SampleTime=Ts_ACR
  Host_Time : DigitalClock  SampleTime=Ts_ACR
  M1A_PWM_Command : FromWorkspace  VariableName=M1A_PWM_ts  SampleTime=Ts_Plant  Interpolate=off  OutputAfterFinalValue=Holding final value
  M1A_Reset_Command : FromWorkspace  VariableName=M1A_Reset_ts  SampleTime=Ts_Plant  Interpolate=off  OutputAfterFinalValue=Holding final value
  M1A_Speed_Command : FromWorkspace  VariableName=M1A_Speed_ts  SampleTime=Ts_Plant  Interpolate=off  OutputAfterFinalValue=Holding final value
  Move_Info_Live_State : DataStoreMemory  DataStoreName=M1B_MoveInfo_Live  InitialValue=zeros(1,8)  ShowAdditionalParam=off
  Move_Info_Vector : Mux
  Move_Ready_Live_State : DataStoreMemory  DataStoreName=M1B_MoveReady_Live  ShowAdditionalParam=off
  Observe_Command_{13..15,18,20..24} (9 alike) : Terminator
  Unused_Host_Environment_Load : Terminator
  Write_Move_Info_Live : DataStoreWrite  DataStoreName=M1B_MoveInfo_Live  IndexOptions=Index vector (dialog)  Indices=1  OutputSizes=1
  Write_Move_Ready_Live : DataStoreWrite  DataStoreName=M1B_MoveReady_Live  IndexOptions=Index vector (dialog)  Indices=1  OutputSizes=1
  x_ref_mm : Outport
  vdc : Outport  Port=2
  Close_Loop_EN : Outport  Port=3
  Position_Loop_EN : Outport  Port=4
  id_ref_cmd : Outport  Port=5
  iq_test_mode : Outport  Port=6
  iq_test_ref : Outport  Port=7
  v_ref_cmd : Outport  Port=8
  PWM_EN : Outport  Port=9
  PI_Reset_EN : Outport  Port=10
  wires:
  Host_Target_mm/1 -> Host_Commands/1
  Host_Speed_mmps/1 -> Host_Commands/2
  Host_Id_A/1 -> Host_Commands/3
  Host_PWM_EN/1 -> Host_Commands/8
  M1A_Speed_Command/1 -> Host_Replay/1
  Host_Iq_Test_Mode/1 -> Host_Commands/4
  Host_Position_Loop_EN/1 -> Host_Commands/6
  M1A_Reset_Command/1 -> Host_Replay/3
  Host_Iq_A/1 -> Host_Commands/5
  Host_Close_Loop_EN/1 -> Host_Commands/7
  Host_PI_Reset_EN/1 -> Host_Commands/9
  Host_Replay_EN/1 -> Host_Commands/10
  Host_Move_Request/1 -> Host_Commands/11
  M1A_PWM_Command/1 -> Host_Replay/2
  alignment_enabled/1 -> Host_Core/5(alignment_enabled)
  Host_Time/1 -> Host_Core/1(t)
  Host_Commands/1 -> Host_Core/2(u)
  Host_Replay/1 -> Host_Core/3(replay)
  Host_Core/5(Position_Loop_EN) -> Position_Loop_EN/1
  x_actual_mm/1 -> Host_Core/4(x_actual_mm)
  Host_Core/4(Close_Loop_EN) -> Close_Loop_EN/1
  alignment_ready/1 -> Host_Core/6(alignment_ready)
  Host_Core/1(x_ref_mm) -> x_ref_mm/1
  Host_Core/2(vdc) -> vdc/1
  Host_Core/3(load_N) -> Unused_Host_Environment_Load/1
  Host_Core/6(PWM_EN) -> PWM_EN/1
  Host_Core/7(v_ref_cmd) -> v_ref_cmd/1
  Host_Core/8(id_ref_cmd) -> id_ref_cmd/1
  Host_Core/9(iq_test_mode) -> iq_test_mode/1
  Host_Core/10(iq_test_ref) -> iq_test_ref/1
  Host_Core/11(PI_Reset_EN) -> PI_Reset_EN/1
  Move_Info_Vector/1 -> Write_Move_Info_Live/1
  Host_Core/13(move_busy) -> Observe_Command_13/1
  Host_Core/14(in_position) -> Observe_Command_14/1
  Host_Core/15(command_status) -> Observe_Command_15/1
  Host_Core/18(trajectory_done) -> Observe_Command_18/1
  Host_Core/20(accepted_count) -> Observe_Command_20/1
  Host_Core/21(rejected_count) -> Observe_Command_21/1
  Host_Core/22(segment_id) -> Observe_Command_22/1
  Host_Core/23(command_received_s) -> Observe_Command_23/1
  Host_Core/24(move_interrupted) -> Observe_Command_24/1
  Host_Core/12(target_accepted_mm) -> [move_target_latched]
  [move_target_latched] -> Move_Info_Vector/2
  Host_Core/16(segment_start_mm) -> [move_segment_start]
  [move_segment_start] -> Move_Info_Vector/1
  Host_Core/17(segment_start_s) -> [move_segment_time]
  [move_segment_time] -> Move_Info_Vector/3
  Host_Core/19(move_ready) -> [move_ready_live]
  [move_ready_live] -> Write_Move_Ready_Live/1
  Host_Core/25(trajectory_config) -> [move_profile_cfg]
  [move_profile_cfg] -> Move_Info_Vector/4

== system PMLSM_PI_FOC_Float_Baseline/Alignment_Interface/Alignment_Angle_Selection ==
  x_mm_in : Inport
  Angle_Init_EN : Inport  Port=2
  Theta_Offset_auto : Inport  Port=3
  Add2 : Sum  Inputs=+++
  Constant4 : Constant  Value=2*pi
  Constant6 : Constant  Value=theta_align_const
  Data Type Conversion : DataTypeConversion  OutDataTypeStr=double  SaturateOnIntegerOverflow=off  RndMeth=Floor
  Gain : Gain  Gain=2*pi/Tau_e_mm
  Math Function1 : Math  Operator=mod
  Switch2 : Switch  Criteria=u2 > Threshold  Threshold=0.5  SaturateOnIntegerOverflow=off  InputSameDT=off
  Theta_Offset : Constant  Value=Theta_Offset_Fine
  etheta : Outport
  wires:
  Gain/1 -> Add2/1
  Theta_Offset_auto/1 -> Add2/2
  Theta_Offset/1 -> Add2/3
  x_mm_in/1 -> Data Type Conversion/1
  Data Type Conversion/1 -> Gain/1
  Angle_Init_EN/1 -> [Angle_Init_EN]
  Add2/1 -> Math Function1/1
  Constant4/1 -> Math Function1/2
  Constant6/1 -> Switch2/1
  [Angle_Init_EN] -> Switch2/2
  Math Function1/1 -> Switch2/3
  Switch2/1 -> etheta/1

== system PMLSM_PI_FOC_Float_Baseline/Alignment_Task_10kHz/Enabled_Original_MIL ==
  Init_Start : Inport
  Init_Reset : Inport  Port=2
  travel_fault_latch : Inport  Port=3
  x_mm : Inport  Port=4
  Enable : EnablePort
  Angle_Init : Stateflow chart  TreatAsAtomicUnit=on
  Init_Done : Outport
  Init_State_Num : Outport  Port=2
  id_init_ref : Outport  Port=3
  Angle_Init_EN : Outport  Port=4
  Theta_Offset_auto : Outport  Port=5
  x_align_mm_latch : Outport  Port=6
  wires:
  Init_Start/1 -> Angle_Init/1(Init_Start)
  Init_Reset/1 -> Angle_Init/2(Init_Reset)
  travel_fault_latch/1 -> Angle_Init/3(travel_fault_latch)
  x_mm/1 -> Angle_Init/4(x_mm)
  Angle_Init/1(Init_Done) -> Init_Done/1  "Init_Done"
  Angle_Init/2(Init_State_Num) -> Init_State_Num/1  "Init_State_Num"
  Angle_Init/3(id_init_ref) -> id_init_ref/1  "id_init_ref"
  Angle_Init/6(x_align_mm_latch) -> x_align_mm_latch/1  "x_align_mm_latch"
  Angle_Init/5(Theta_Offset_auto) -> Theta_Offset_auto/1  "Theta_Offset_auto"
  Angle_Init/4(Angle_Init_EN) -> Angle_Init_EN/1  "Angle_Init_EN"

== system PMLSM_PI_FOC_Float_Baseline/Control_Task_10kHz/FOC_Implementation ==
  ia : Inport
  ib : Inport  Port=2
  ic : Inport  Port=3
  theta_e : Inport  Port=4
  omega_e : Inport  Port=5
  iq_ref : Inport  Port=6
  id_ref : Inport  Port=7
  PI_Reset_EN : Inport  Port=8
  Vdc_V : Inport  Port=9
  Fixed : Subsystem  VariantControl=FOC_Impl_Select == 1
  Float : Subsystem  VariantControl=FOC_Impl_Select == 0
  duty_u_cmd : Outport
  duty_v_cmd : Outport  Port=2
  duty_w_cmd : Outport  Port=3

== system PMLSM_PI_FOC_Float_Baseline/Control_Task_10kHz/Position_Loop ==
  x_ref_mm : Inport
  x_mm : Inport  Port=2
  pos_pi_reset : Inport  Port=3
  v_ff_pos : Inport  Port=4
  Trigger : TriggerPort  VariantControl=(inherit)
  Dead Zone : DeadZone  LowerValue=-Pos_deadband  UpperValue=+Pos_deadband
  Gain : Gain  Gain=Kp_pos
  Saturation : Saturate  UpperLimit=V_pos_max_mmps  LowerLimit=-V_pos_max_mmps
  Sum : Sum  Inputs=|+-
  Sum1 : Sum  Inputs=|++
  Terminator : Terminator
  v_ref_pos : Outport
  wires:
  x_ref_mm/1 -> Sum/1
  x_mm/1 -> Sum/2
  Sum/1 -> Dead Zone/1  "e_pos"
  Dead Zone/1 -> Gain/1
  Gain/1 -> Sum1/1
  v_ff_pos/1 -> Sum1/2
  Sum1/1 -> Saturation/1
  pos_pi_reset/1 -> Terminator/1
  Saturation/1 -> v_ref_pos/1  "obs_v_ref_pos"

== system PMLSM_PI_FOC_Float_Baseline/Control_Task_10kHz/Reference_Manager ==
  iq_ref_normal : Inport
  v_ref_pos : Inport  Port=2
  Pos_Loop_EN : Inport  Port=3
  Close_Loop_EN : Inport  Port=4
  v_ref_cmd : Inport  Port=5
  id_ref_cmd : Inport  Port=6
  Iq_Test_Mode : Inport  Port=7
  iq_test_ref : Inport  Port=8
  Constant15 : Constant  Value=0
  Saturation : Saturate  UpperLimit=v_ref_max  LowerLimit=-v_ref_max
  Switch : Switch  Criteria=u2 > Threshold  Threshold=0.5  SaturateOnIntegerOverflow=off  InputSameDT=off
  Switch9 : Switch  Criteria=u2 > Threshold  Threshold=0.5  SaturateOnIntegerOverflow=off  InputSameDT=off
  v_ref_closed_sel : Switch  Criteria=u2 > Threshold  Threshold=0.5  SaturateOnIntegerOverflow=off  InputSameDT=off
  v_ref_set_slew_limiter : Subsystem
  id_ref : Outport
  iq_ref : Outport  Port=2
  v_ref : Outport  Port=3
  wires:
  Switch/1 -> iq_ref/1
  Switch9/1 -> v_ref/1
  Close_Loop_EN/1 -> Switch9/2
  iq_test_ref/1 -> Switch/1
  Iq_Test_Mode/1 -> Switch/2
  Constant15/1 -> Switch9/3
  iq_ref_normal/1 -> Switch/3
  id_ref_cmd/1 -> id_ref/1
  v_ref_set_slew_limiter/1(v_ref_set_limited) -> Saturation/1
  v_ref_pos/1 -> v_ref_closed_sel/1
  v_ref_closed_sel/1 -> v_ref_set_slew_limiter/1(v_ref_set)  "v_ref_closed"
  Pos_Loop_EN/1 -> v_ref_closed_sel/2
  Saturation/1 -> Switch9/1
  v_ref_cmd/1 -> v_ref_closed_sel/3

== system PMLSM_PI_FOC_Float_Baseline/Control_Task_10kHz/Scheduler_10k_1k_100 ==
  note: position 计数链(/100)
  note: speed 计数链(/10)
  Add1 : Sum
  Add2 : Sum
  Constant1 : Constant
  Constant2 : Constant  Value=0
  Constant3 : Constant
  Constant4 : Constant  Value=0
  Logical Operator : Logic  AllPortsSameDT=off  OutDataTypeStr=boolean
  pos_cnt_hold_sel : Switch  Criteria=u2 > Threshold  Threshold=0.5  SaturateOnIntegerOverflow=off  InputSameDT=off
  pos_cnt_update_sel : Switch  Criteria=u2 > Threshold  Threshold=0.5  SaturateOnIntegerOverflow=off  InputSameDT=off
  pos_cnt_z : UnitDelay  SampleTime=-1
  pos_tc : simulink/Logic and Bit Operations/Compare To Constant  relop=>=  const=10  OutDataTypeStr=boolean
  spd_cnt_next_sel : Switch  Criteria=u2 > Threshold  Threshold=0.5  SaturateOnIntegerOverflow=off  InputSameDT=off
  spd_cnt_z : UnitDelay  SampleTime=-1
  spd_tc : simulink/Logic and Bit Operations/Compare To Constant  relop=>=  const=10  OutDataTypeStr=boolean
  speed_tick : Outport
  pos_tick : Outport  Port=2
  wires:
  spd_cnt_z/1 -> Add1/1
  spd_tc/1 -> speed_tick/1, Logical Operator/1, pos_cnt_hold_sel/2, spd_cnt_next_sel/2
  Constant1/1 -> Add1/2
  Constant2/1 -> spd_cnt_next_sel/1
  spd_cnt_next_sel/1 -> spd_cnt_z/1
  Add1/1 -> spd_cnt_next_sel/3, spd_tc/1  "spd_cnt_inc"
  pos_cnt_z/1 -> Add2/1, pos_cnt_hold_sel/3
  Constant3/1 -> Add2/2
  Add2/1 -> pos_cnt_update_sel/3, pos_tc/1  "pos_cnt_inc"
  pos_tc/1 -> Logical Operator/2, pos_cnt_update_sel/2
  Constant4/1 -> pos_cnt_update_sel/1
  pos_cnt_update_sel/1 -> pos_cnt_hold_sel/1  "pos_cnt_update_candidate"
  pos_cnt_hold_sel/1 -> pos_cnt_z/1
  Logical Operator/1 -> pos_tick/1

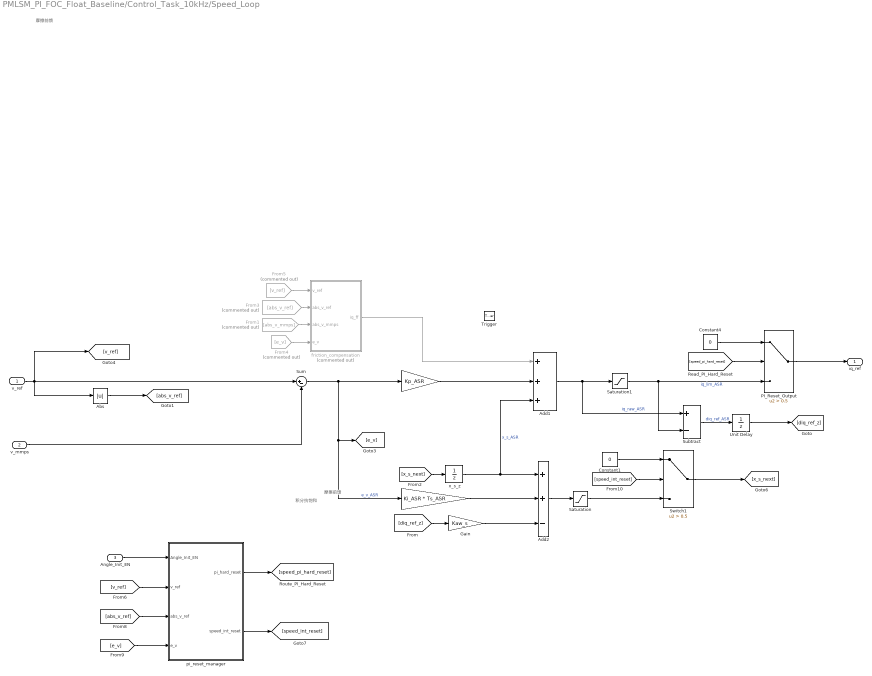
== system PMLSM_PI_FOC_Float_Baseline/Control_Task_10kHz/Speed_Loop ==
  note: 摩擦前馈
  note: 积分抗饱和
  note: 摩擦前馈
  v_ref : Inport
  v_mmps : Inport  Port=2
  Angle_Init_EN : Inport  Port=3
  Trigger : TriggerPort  VariantControl=(inherit)
  " " : Gain  Gain=Ki_ASR * Ts_ASR
  "  " : Gain  Gain=Kp_ASR
  Abs : Abs  SaturateOnIntegerOverflow=off
  Add1 : Sum  Inputs=+++
  Add2 : Sum  Inputs=++-
  Constant1 : Constant  Value=0
  Constant4 : Constant  Value=0
  From1 : From  Commented=on  GotoTag=abs_v_mmps
  From3 : From  Commented=on  GotoTag=abs_v_ref
  From4 : From  Commented=on  GotoTag=e_v
  From5 : From  Commented=on  GotoTag=v_ref
  Gain : Gain  Gain=Kaw_s
  PI_Reset_Output : Switch  Criteria=u2 > Threshold  Threshold=0.5  SaturateOnIntegerOverflow=off  InputSameDT=off
  Saturation : Saturate  UpperLimit=Iq_int_limit  LowerLimit=-Iq_int_limit
  Saturation1 : Saturate  UpperLimit=Speed_loop_Iq_Limit  LowerLimit=-Speed_loop_Iq_Limit
  Subtract : Sum  Inputs=+-
  Sum : Sum  Inputs=|+-
  Switch1 : Switch  Criteria=u2 > Threshold  Threshold=0.5  SaturateOnIntegerOverflow=off  InputSameDT=off
  Unit Delay : UnitDelay  SampleTime=-1
  friction_compensation : Subsystem  Commented=on
  pi_reset_manager : Subsystem
  x_s_z : UnitDelay  SampleTime=-1
  iq_ref : Outport
  wires:
  Sum/1 -> [e_v], " "/1, "  "/1  "e_v_ASR"
  Add1/1 -> Subtract/1, Saturation1/1  "iq_raw_ASR"
  v_ref/1 -> Sum/1, Abs/1, [v_ref]
  Saturation1/1 -> PI_Reset_Output/3, Subtract/2  "iq_lim_ASR"
  [x_s_next] -> x_s_z/1
  Add2/1 -> Saturation/1
  Gain/1 -> Add2/3
  " "/1 -> Add2/2
  Subtract/1 -> Unit Delay/1  "diq_ref_ASR"
  Unit Delay/1 -> [diq_ref_z]
  [diq_ref_z] -> Gain/1
  Constant1/1 -> Switch1/1
  PI_Reset_Output/1 -> iq_ref/1
  Constant4/1 -> PI_Reset_Output/1
  "  "/1 -> Add1/2
  friction_compensation/1(iq_ff) -> Add1/1
  x_s_z/1 -> Add1/3, Add2/1  "x_s_ASR"
  From4/1 -> friction_compensation/4(e_v)
  From1/1 -> friction_compensation/3(abs_v_mmps)
  From3/1 -> friction_compensation/2(abs_v_ref)
  Abs/1 -> [abs_v_ref]
  Angle_Init_EN/1 -> pi_reset_manager/1(Angle_Init_EN)
  From5/1 -> friction_compensation/1(v_ref)
  [v_ref] -> pi_reset_manager/2(v_ref)
  [abs_v_ref] -> pi_reset_manager/3(abs_v_ref)
  [e_v] -> pi_reset_manager/4(e_v)
  [speed_pi_hard_reset] -> PI_Reset_Output/2
  pi_reset_manager/2(speed_int_reset) -> [speed_int_reset]
  pi_reset_manager/1(pi_hard_reset) -> [speed_pi_hard_reset]
  [speed_int_reset] -> Switch1/2
  Switch1/1 -> [x_s_next]
  Saturation/1 -> Switch1/3
  v_mmps/1 -> Sum/2

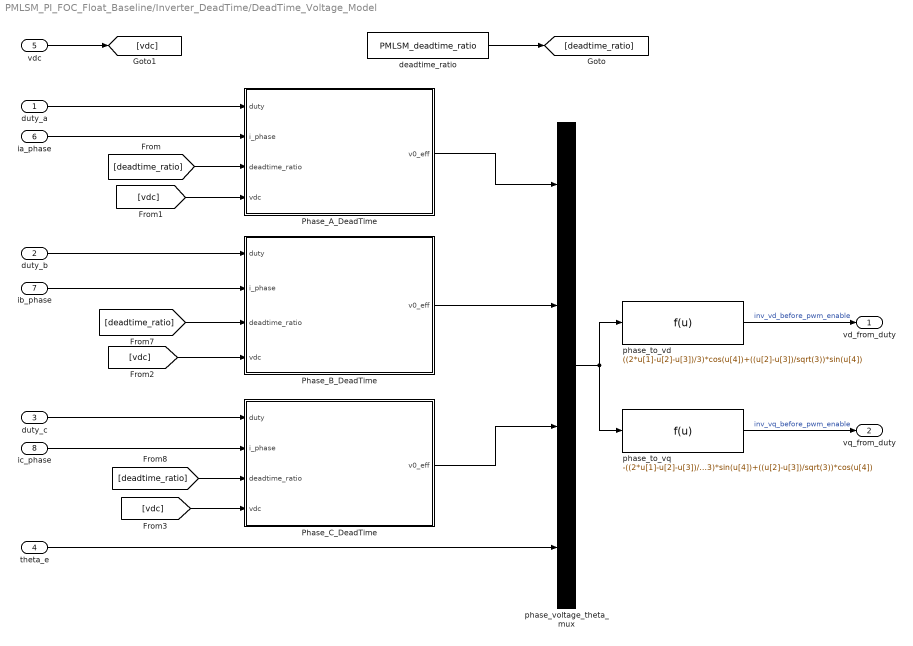
== system PMLSM_PI_FOC_Float_Baseline/Inverter_DeadTime/DeadTime_Voltage_Model ==
  duty_a : Inport
  duty_b : Inport  Port=2
  duty_c : Inport  Port=3
  theta_e : Inport  Port=4
  vdc : Inport  Port=5
  ia_phase : Inport  Port=6
  ib_phase : Inport  Port=7
  ic_phase : Inport  Port=8
  Phase_A_DeadTime : Subsystem
  Phase_B_DeadTime : Subsystem
  Phase_C_DeadTime : Subsystem
  deadtime_ratio : Constant  Value=PMLSM_deadtime_ratio
  phase_to_vd : Fcn  Expr=((2*u[1]-u[2]-u[3])/3)*cos(u[4])+((u[2]-u[3])/sqrt(3))*sin(u[4])
  phase_to_vq : Fcn  Expr=-((2*u[1]-u[2]-u[3])/3)*sin(u[4])+((u[2]-u[3])/sqrt(3))*cos(u[4])
  phase_voltage_theta_mux : Mux
  vd_from_duty : Outport
  vq_from_duty : Outport  Port=2
  wires:
  [deadtime_ratio] -> Phase_C_DeadTime/3(deadtime_ratio)
  [deadtime_ratio] -> Phase_B_DeadTime/3(deadtime_ratio)
  [deadtime_ratio] -> Phase_A_DeadTime/3(deadtime_ratio)
  [vdc] -> Phase_C_DeadTime/4(vdc)
  [vdc] -> Phase_B_DeadTime/4(vdc)
  [vdc] -> Phase_A_DeadTime/4(vdc)
  vdc/1 -> [vdc]
  theta_e/1 -> phase_voltage_theta_mux/4
  Phase_C_DeadTime/1(v0_eff) -> phase_voltage_theta_mux/3
  Phase_B_DeadTime/1(v0_eff) -> phase_voltage_theta_mux/2
  Phase_A_DeadTime/1(v0_eff) -> phase_voltage_theta_mux/1
  ic_phase/1 -> Phase_C_DeadTime/2(i_phase)
  duty_c/1 -> Phase_C_DeadTime/1(duty)
  ib_phase/1 -> Phase_B_DeadTime/2(i_phase)
  duty_b/1 -> Phase_B_DeadTime/1(duty)
  ia_phase/1 -> Phase_A_DeadTime/2(i_phase)
  duty_a/1 -> Phase_A_DeadTime/1(duty)
  deadtime_ratio/1 -> [deadtime_ratio]
  phase_to_vq/1 -> vq_from_duty/1  "inv_vq_before_pwm_enable"
  phase_to_vd/1 -> vd_from_duty/1  "inv_vd_before_pwm_enable"
  phase_voltage_theta_mux/1 -> phase_to_vq/1, phase_to_vd/1

== system PMLSM_PI_FOC_Float_Baseline/Inverter_DeadTime/PWM_Update_HalfTs ==
  duty_a : Inport
  duty_b : Inport  Port=2
  duty_c : Inport  Port=3
  a_cmd_zoh : ZeroOrderHold  SampleTime=Ts
  a_half_Ts : UnitDelay  InitialCondition=0.5  SampleTime=M1A_PWM_Update_Delay_s
  b_cmd_zoh : ZeroOrderHold  SampleTime=Ts
  b_half_Ts : UnitDelay  InitialCondition=0.5  SampleTime=M1A_PWM_Update_Delay_s
  c_cmd_zoh : ZeroOrderHold  SampleTime=Ts
  c_half_Ts : UnitDelay  InitialCondition=0.5  SampleTime=M1A_PWM_Update_Delay_s
  duty_a_delayed : Outport
  duty_b_delayed : Outport  Port=2
  duty_c_delayed : Outport  Port=3
  wires:
  duty_c/1 -> c_cmd_zoh/1
  duty_b/1 -> b_cmd_zoh/1
  duty_a/1 -> a_cmd_zoh/1
  c_half_Ts/1 -> duty_c_delayed/1
  b_half_Ts/1 -> duty_b_delayed/1
  a_half_Ts/1 -> duty_a_delayed/1
  a_cmd_zoh/1 -> a_half_Ts/1
  b_cmd_zoh/1 -> b_half_Ts/1
  c_cmd_zoh/1 -> c_half_Ts/1

== system PMLSM_PI_FOC_Float_Baseline/Control_Task_10kHz/FOC_Implementation/Fixed ==
  ia : Inport
  ib : Inport  Port=2
  ic : Inport  Port=3
  theta_e : Inport  Port=4
  omega_e : Inport  Port=5
  iq_ref : Inport  Port=6
  id_ref : Inport  Port=7
  PI_Reset_EN : Inport  Port=8
  Vdc_V : Inport  Port=9
  Decode_Duty1 : DataTypeConversion  OutDataTypeStr=double
  Decode_Duty2 : DataTypeConversion  OutDataTypeStr=double
  Decode_Duty3 : DataTypeConversion  OutDataTypeStr=double
  Encode_PI_Reset_EN : DataTypeConversion  OutDataTypeStr=boolean  RndMeth=Convergent
  Encode_Vdc_V : DataTypeConversion  OutDataTypeStr=FOC_Fixed_Config.Types.Bus  RndMeth=Convergent
  Encode_ia : DataTypeConversion  OutDataTypeStr=FOC_Fixed_Config.Types.Current  RndMeth=Convergent
  Encode_ib : DataTypeConversion  OutDataTypeStr=FOC_Fixed_Config.Types.Current  RndMeth=Convergent
  Encode_ic : DataTypeConversion  OutDataTypeStr=FOC_Fixed_Config.Types.Current  RndMeth=Convergent
  Encode_id_ref : DataTypeConversion  OutDataTypeStr=FOC_Fixed_Config.Types.Current  RndMeth=Convergent
  Encode_iq_ref : DataTypeConversion  OutDataTypeStr=FOC_Fixed_Config.Types.Current  RndMeth=Convergent
  Encode_omega_e : DataTypeConversion  OutDataTypeStr=FOC_Fixed_Config.Types.Omega  RndMeth=Convergent
  Encode_theta_e : DataTypeConversion  OutDataTypeStr=FOC_Fixed_Config.Types.Angle  RndMeth=Convergent
  FOC_Model : ModelReference  ModelNameDialog=PMLSM_FOC_FixedPoint  SimulationMode=Normal  ModelReferenceVersion=1.14
  duty_u_cmd : Outport
  duty_v_cmd : Outport  Port=2
  duty_w_cmd : Outport  Port=3
  wires:
  Decode_Duty1/1 -> duty_u_cmd/1
  Decode_Duty2/1 -> duty_v_cmd/1
  Decode_Duty3/1 -> duty_w_cmd/1
  FOC_Model/3 -> Decode_Duty3/1
  FOC_Model/2 -> Decode_Duty2/1
  FOC_Model/1 -> Decode_Duty1/1
  Encode_Vdc_V/1 -> FOC_Model/9
  Encode_omega_e/1 -> FOC_Model/5
  Encode_iq_ref/1 -> FOC_Model/6
  Encode_id_ref/1 -> FOC_Model/7
  Encode_PI_Reset_EN/1 -> FOC_Model/8
  Encode_ib/1 -> FOC_Model/2
  Encode_ic/1 -> FOC_Model/3
  Encode_theta_e/1 -> FOC_Model/4
  Encode_ia/1 -> FOC_Model/1
  PI_Reset_EN/1 -> Encode_PI_Reset_EN/1
  id_ref/1 -> Encode_id_ref/1
  iq_ref/1 -> Encode_iq_ref/1
  Vdc_V/1 -> Encode_Vdc_V/1
  omega_e/1 -> Encode_omega_e/1
  theta_e/1 -> Encode_theta_e/1
  ic/1 -> Encode_ic/1
  ib/1 -> Encode_ib/1
  ia/1 -> Encode_ia/1

== system PMLSM_PI_FOC_Float_Baseline/Control_Task_10kHz/FOC_Implementation/Float ==
  ia : Inport
  ib : Inport  Port=2
  ic : Inport  Port=3
  theta_e : Inport  Port=4
  omega_e : Inport  Port=5
  iq_ref : Inport  Port=6
  id_ref : Inport  Port=7
  PI_Reset_EN : Inport  Port=8
  Vdc_V : Inport  Port=9
  FOC_Algorithm : Subsystem
  Original_Udc_Base_Reference : Terminator
  duty_u_cmd : Outport
  duty_v_cmd : Outport  Port=2
  duty_w_cmd : Outport  Port=3
  wires:
  ia/1 -> FOC_Algorithm/1(ia)
  ic/1 -> FOC_Algorithm/3(ic)
  ib/1 -> FOC_Algorithm/2(ib)
  FOC_Algorithm/1(duty_u_cmd) -> duty_u_cmd/1
  FOC_Algorithm/3(duty_w_cmd) -> duty_w_cmd/1
  theta_e/1 -> FOC_Algorithm/4(theta_e)
  iq_ref/1 -> FOC_Algorithm/6(iq_ref)
  omega_e/1 -> FOC_Algorithm/5(omega_e)
  FOC_Algorithm/2(duty_v_cmd) -> duty_v_cmd/1
  id_ref/1 -> FOC_Algorithm/7(id_ref)
  PI_Reset_EN/1 -> FOC_Algorithm/8(PI_Reset_EN)
  Vdc_V/1 -> Original_Udc_Base_Reference/1

== system PMLSM_PI_FOC_Float_Baseline/Control_Task_10kHz/Reference_Manager/v_ref_set_slew_limiter ==
  v_ref_set : Inport
  Add : Sum
  Saturation : Saturate  UpperLimit=v_ref_set_step_up  LowerLimit=-v_ref_set_step_dn
  Subtract : Sum  Inputs=+-
  v_ref_set_lim_z : UnitDelay  SampleTime=-1
  v_ref_set_limited : Outport
  wires:
  v_ref_set_lim_z/1 -> Add/2, Subtract/2
  v_ref_set/1 -> Subtract/1
  Saturation/1 -> Add/1
  Subtract/1 -> Saturation/1
  Add/1 -> v_ref_set_limited/1, v_ref_set_lim_z/1
